simulink model "PassVeh14DOF"  (R2026b)
settings: Solver=ode23tb  StopTime=inf  FixedStep=.001  RelTol=1e-1  EnableMultiTasking=on
model workspace (MAT data in the model file):
  AlgnTrqCambCompl = [0 0 0 0]
  AlgnTrqSteerCompl = [0 0 0 0]
  AxlIxx = 62.3745166667
  AxlM = 160
  BumpCamber = [0 0 0 0]
  BumpCaster = [0 0 0 0]
  BumpSteer = [0 0 0 0]
  CambVsSteerAng = [0 0 0 0]
  CastVsSteerAng = [0 0 0 0]
  Cps = 2
  Cz = 5565.2246438
  CzWhlAxl = 11490.971257
  DCT_Param : object (value not decoded)
  Downshift_Speeds = [9.5625 12.9375 16.3125 19.6875 23.0625 26.4375 29.8125 33.1875 36.5625 39.9375 43.3125 46.6875 ... (28 elements, 4x7)]
  F0z = [2886 2907]
  F0zWhlAxl = 2907
  Hmax = 0.25
  Kz = 52451.0065793
  KzWhlAxl = 138031.612078
  LatCambCompl = [0 0 0 0]
  LatSteerCompl = [0 0 0 0]
  LatWhlCtrComplLat = [0 0 0 0]
  LatWhlCtrComplLng = [0  0  0  0; 0  0  0  0]
  LatWhlCtrDisp = [0 0 0 0]
  LngCambCompl = [0  0  0  0; 0  0  0  0]
  LngCastCompl = [0  0  0  0; 0  0  0  0]
  LngSteerCompl = [0  0  0  0; 0  0  0  0]
  LngWhlCtrCompl = [0  0  0  0; 0  0  0  0]
  LngWhlCtrDisp = [0 0 0 0]
  MotRatios = [1 1]
  NCyl = 6
  NrmlWhlFrcOff = [2886 2886 2907 2907]
  NrmlWhlRates = [52.4510065793 52.4510065793 52.4510065793 52.4510065793]
  Pedal_Positions = [0.1 0.4 0.5 0.9]
  Pstd = 101325
  Rair = 287
  RollCamber : object (value not decoded)
  RollCaster : object (value not decoded)
  RollSteer : object (value not decoded)
  RollStiffArb = [0 0]
  RollStiffArbFrnt = 800
  RollStiffNoArb = [0 0]
  RollStiffNoArbFrnt = 0
  RollStiffNoTwstRear = 0
  ShckFrcVsCompRate = [5.5652246438 5.5652246438 5.5652246438 5.5652246438]
  StatCamber = [0 0 0 0]
  StatCaster = [0 0 0 0]
  StatLdWhlR = [0.3 0.3 0.3 0.3]
  StatToe = [0 0 0 0]
  Trans : object (value not decoded)
  Tstd = 293.15
  Upshift_Speeds = [12.9375 16.3125 19.6875 33 26.4375 29.8125 33.1875 52.5 39.9375 43.3125 46.6875 77.25 ... (28 elements, 4x7)]
  VEH : object (value not decoded)
  Vd = 0.00346
  VrtLdTrnsfr = [0 0 0 0]
  WH : Mass (value not decoded)
  dt3D = 0.05
  f_air = [0 0 0 0 0 0 0 0 0 0 0 0 ... (256 elements, 16x16)]
  f_co = [0 0 0 0 0 0 0 0 0 0 0 0 ... (256 elements, 16x16)]
  f_co2 = [0 0 0 0 0 0 0 0 0 0 0 0 ... (256 elements, 16x16)]
  f_eff = [352.135682859 352.135682859 320.724378192 303.655312657 295.930136708 291.240087194 291.240271258 291.240312459 291.240275452 291.240198499 291.240100781 291.240018769 ... (256 elements, 16x16)]
  f_fuel = [0 0 0 0 0 0 0 0 0 0 0 0 ... (256 elements, 16x16)]
  f_hc = [0 0 0 0 0 0 0 0 0 0 0 0 ... (256 elements, 16x16)]
  f_nox = [0 0 0 0 0 0 0 0 0 0 0 0 ... (256 elements, 16x16)]
  f_pm = [0 0 0 0 0 0 0 0 0 0 0 0 ... (256 elements, 16x16)]
  f_susp_axl_bp = [1 2]
  f_susp_dz_bp = [-0.325022776267 -0.315022776267 -0.305022776267 -0.205022776267 -0.105022776267 -0.00502277626717 0.0949772237328 0.194977223733 0.204977223733 0.214977223733]
  f_susp_dzdot_bp = [-3 -0.3 -0.2 -0.1 0 0.1 0.2 0.3 3]
  f_susp_fmz = [-144070.391448 -93629.24037 -75929.1118915 -20630.5828179 -15385.48216 -10140.3815021 -4895.28084414 349.819813785 -31916.3973792 18437.6709544 -83996.1993354 -33555.0482577 ... (43920 elements, 10x9x61x2x4)]
  f_susp_geom = [0 0 0 0 0 0 0 0 0 0 0 0 ... (3660 elements, 10x61x2x3)]
  f_susp_strgdelta_bp = [-0.523598775598 -0.506145483078 -0.488692190558 -0.471238898038 -0.453785605519 -0.436332312999 -0.418879020479 -0.401425727959 -0.383972435439 -0.366519142919 -0.349065850399 -0.331612557879 ... (61 elements, 1x61)]
  f_tbrake = [0 76.8593923996 105.140482948 131.533638111 157.926793274 176.658631717 176.65727296 176.656856686 176.656879077 176.657093756 176.657404516 176.65772406 ... (256 elements, 16x16)]
  f_tbrake_n_bpt = [0 649.519052838 912.419621844 1175.32019085 1438.22075986 1701.12132886 1964.02189787 2226.92246687 2489.82303588 2752.72360489 3015.62417389 3278.5247429 ... (16 elements, 1x16)]
  f_tbrake_t_bpt = [0 34.6410161514 61.0341713143 87.4273264773 113.82048164 140.213636803 166.606791966 192.999947129 219.393102292 245.786257455 272.179412618 298.572567781 ... (16 elements, 1x16)]
  f_texh = [766.752464599 766.752464599 786.17542386 801.679939032 884.591982581 910.574397722 910.571871054 910.570774534 910.570601632 910.570821151 910.571247242 910.571639815 ... (256 elements, 16x16)]
  f_twc_eff_co = [0.17 0.25 0.45 0.99 0.99 0.99 0.99]
  f_twc_eff_hc = [0.21 0.375 0.75 0.98 0.98 0.98 0.98]
  f_twc_eff_lam = [0.909090909 0.944055944 0.979020979 1 1.013986014 1.048951049 1.083916084]
  f_twc_eff_nox = [0.98 0.98 0.98 0.97 0.05 0.02 0]
  numWheel = 4
symbols that are objects in the model workspace (value not decoded): VEH
libraries: vehdynlibtire x12, vehdynlibsuspension x8, autolibutils x5, sharedtransform x5, shared6dof x2, vehdynlibeom x1, vehdynlibtirecommon x1, matrix_library x1
(part 4 of 9)

== system PassVeh14DOF/Vehicle/Suspension to Chasiss Transforms/Susp2Body ==
  DCM : Inport
  VehAng : Inport  Port=2
  SuspAng : Inport  Port=3
  Fs : Inport  Port=4  Partition=on  PartitionDimension=2  PartitionWidth=1  PartitionOffset=0
  Ms : Inport  Port=5  Partition=on  PartitionDimension=2  PartitionWidth=1  PartitionOffset=0
  For Each : ForEach  DisableCoverage=on
  Inertial to Body : Product  Multiplication=Matrix(*)  InputSameDT=on  SaturateOnIntegerOverflow=on  OutDataTypeStr=Inherit: Same as first input
  Inertial to Body1 : Product  Multiplication=Matrix(*)  InputSameDT=on  SaturateOnIntegerOverflow=on  OutDataTypeStr=Inherit: Same as first input
  Reshape : Reshape
  Reshape1 : Reshape
  Rotation Angles to Direction Cosine Matrix : sharedtransform/Rotation Angles to Direction Cosine Matrix  rotationOrder=ZYX  aMode=2
  Selector : Selector  InputPortWidth=3  IndexOptions=Index vector (dialog)  Indices=[3 2 1]  OutputSizes=1
  Selector1 : Selector  InputPortWidth=3  IndexOptions=Index vector (dialog)  Indices=[1 2]  OutputSizes=1
  Selector2 : Selector  InputPortWidth=3  IndexOptions=Index vector (dialog)  Indices=[3]  OutputSizes=1
  Transpose : Math  Operator=transpose  SignedPower=on
  Unary Minus : UnaryMinus
  Vector Concatenate : Concatenate
  "transform to Inertial axes " : shared6dof/6DOF (Euler Angles)/transform to Inertial axes   SystemSampleTime=-1  VariantActivationTime=update diagram  EmptyChoice=off  PassThrough=off  PassThroughVariantControl=(default)  EmptyChoiceVariantControl=(default)  AllowFlexibleInterface=on  Latency=0  AutoFrameSizeCalculation=off
  transform to Inertial axes 1 : shared6dof/6DOF (Euler Angles)/transform to Inertial axes   SystemSampleTime=-1  VariantActivationTime=update diagram  EmptyChoice=off  PassThrough=off  PassThroughVariantControl=(default)  EmptyChoiceVariantControl=(default)  AllowFlexibleInterface=on  Latency=0  AutoFrameSizeCalculation=off
  FsB : Outport  ConcatenationDimension=2  VectorParamsAs1DForOutWhenUnconnected=off
  MsB : Outport  Port=2  ConcatenationDimension=2  VectorParamsAs1DForOutWhenUnconnected=off
  wires:
  Reshape/1 -> Inertial to Body/2
  Inertial to Body/1 -> FsB/1
  SuspAng/1 -> Unary Minus/1
  Selector/1 -> Rotation Angles to Direction Cosine Matrix/1
  Fs/1 -> "transform to Inertial axes "/1
  Transpose/1 -> transform to Inertial axes 1/2, "transform to Inertial axes "/2
  Rotation Angles to Direction Cosine Matrix/1 -> Transpose/1
  "transform to Inertial axes "/1 -> Reshape/1
  transform to Inertial axes 1/1 -> Reshape1/1
  Inertial to Body1/1 -> MsB/1
  Reshape1/1 -> Inertial to Body1/2
  DCM/1 -> Inertial to Body1/1, Inertial to Body/1
  Ms/1 -> transform to Inertial axes 1/1
  VehAng/1 -> Selector2/1
  Unary Minus/1 -> Selector1/1
  Selector1/1 -> Vector Concatenate/1
  Vector Concatenate/1 -> Selector/1
  Selector2/1 -> Vector Concatenate/2

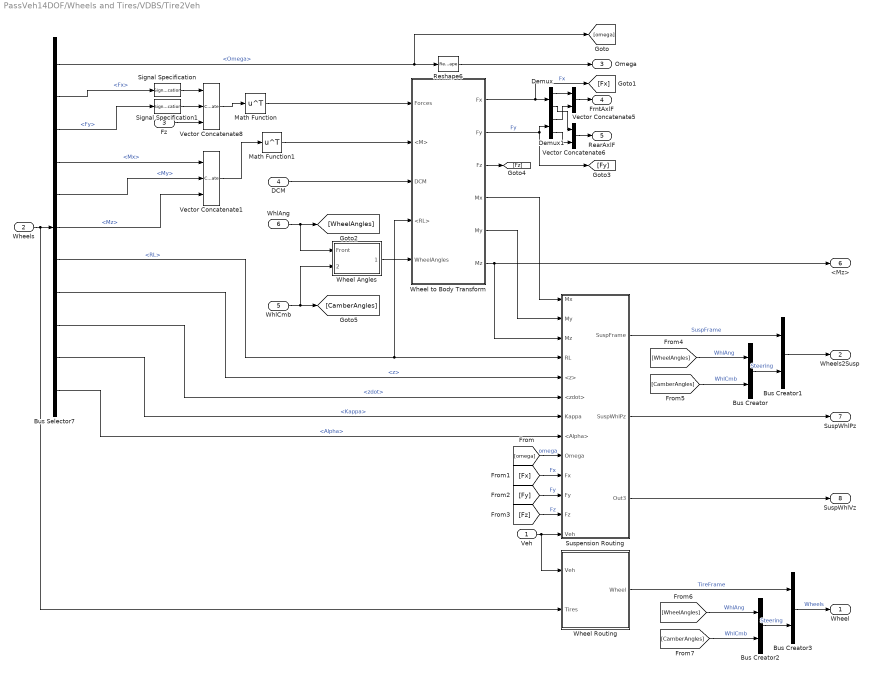
== system PassVeh14DOF/Wheels and Tires/VDBS/Tire2Veh ==
  Veh : Inport
  Wheels : Inport  Port=2
  Fz : Inport  Port=3  PortDimensions=4
  DCM : Inport  Port=4
  WhlCmb : Inport  Port=5
  WhlAng : Inport  Port=6
  Bus Creator{,1..3} (4 alike) : BusCreator  Inputs=2
  Bus Selector7 : BusSelector  OutputSignals=Omega,Fx,Fy,Mx,My,Mz,RL,z,zdot,Kappa,Alpha
  Demux : Demux  Outputs=[2,2]
  Demux1 : Demux  Outputs=[2,2]
  Math Function : Math  Operator=transpose  SignedPower=on
  Math Function1 : Math  Operator=transpose  SignedPower=on
  Reshape6 : Reshape  OutputDimensionality=Customize  OutputDimensions=[2,2]
  Signal Specification : SignalSpecification  Dimensions=4
  Signal Specification1 : SignalSpecification  Dimensions=4
  Suspension Routing : Subsystem
  Vector Concatenate1 : Concatenate  NumInputs=3  Mode=Multidimensional array  ConcatenateDimension=2
  Vector Concatenate5 : Concatenate  Mode=Multidimensional array  ConcatenateDimension=2
  Vector Concatenate6 : Concatenate  Mode=Multidimensional array  ConcatenateDimension=2
  Vector Concatenate8 : Concatenate  NumInputs=3  Mode=Multidimensional array  ConcatenateDimension=2
  Wheel Angles : Subsystem
  Wheel Routing : Subsystem
  Wheel to Body Transform : Subsystem
  Wheel : Outport  VectorParamsAs1DForOutWhenUnconnected=off
  Wheels2Susp : Outport  Port=2  VectorParamsAs1DForOutWhenUnconnected=off
  Omega : Outport  Port=3  VectorParamsAs1DForOutWhenUnconnected=off
  FrntAxlF : Outport  Port=4  VectorParamsAs1DForOutWhenUnconnected=off
  RearAxlF : Outport  Port=5  VectorParamsAs1DForOutWhenUnconnected=off
  <Mz> : Outport  Port=6  VectorParamsAs1DForOutWhenUnconnected=off
  SuspWhlPz : Outport  Port=7  VectorParamsAs1DForOutWhenUnconnected=off
  SuspWhlVz : Outport  Port=8  VectorParamsAs1DForOutWhenUnconnected=off
  wires:
  Fz/1 -> Vector Concatenate8/3
  Vector Concatenate6/1 -> RearAxlF/1
  Vector Concatenate8/1 -> Math Function/1
  Demux/2 -> Vector Concatenate6/1
  Demux1/2 -> Vector Concatenate6/2
  Demux/1 -> Vector Concatenate5/1
  Math Function/1 -> Wheel to Body Transform/1(Forces)
  Bus Selector7/2 -> Signal Specification/1  "<Fx>"
  Vector Concatenate5/1 -> FrntAxlF/1
  Wheels/1 -> Wheel Routing/2(Tires), Bus Selector7/1
  Reshape6/1 -> Omega/1
  Demux1/1 -> Vector Concatenate5/2
  Wheel Angles/1(Vehicle) -> Wheel to Body Transform/5(WheelAngles)
  Bus Selector7/1 -> [omega], Reshape6/1  "<Omega>"
  WhlAng/1 -> Wheel Angles/1(Front), [WheelAngles]
  Wheel to Body Transform/3(Fz) -> [Fz]
  WhlCmb/1 -> Wheel Angles/2(Camber), [CamberAngles]
  Bus Selector7/3 -> Signal Specification1/1  "<Fy>"
  Bus Selector7/5 -> Vector Concatenate1/2  "<My>"
  [omega] -> Suspension Routing/9(Omega)  "omega"
  [Fx] -> Suspension Routing/10(Fx)  "Fx"
  Bus Selector7/8 -> Suspension Routing/5(<z>)  "<z>"
  [Fy] -> Suspension Routing/11(Fy)  "Fy"
  [Fz] -> Suspension Routing/12(Fz)  "Fz"
  Bus Selector7/9 -> Suspension Routing/6(<zdot>)  "<zdot>"
  Bus Selector7/10 -> Suspension Routing/7(Kappa)  "<Kappa>"
  Suspension Routing/2(SuspWhlPz) -> SuspWhlPz/1
  Suspension Routing/3(Out3) -> SuspWhlVz/1
  [WheelAngles] -> Bus Creator/1  "WhlAng"
  Bus Creator1/1 -> Wheels2Susp/1
  Suspension Routing/1(SuspFrame) -> Bus Creator1/1  "SuspFrame"
  [CamberAngles] -> Bus Creator/2  "WhlCmb"
  Bus Creator/1 -> Bus Creator1/2  "Steering"
  Bus Selector7/11 -> Suspension Routing/8(<Alpha>)  "<Alpha>"
  Wheel to Body Transform/1(Fx) -> [Fx], Demux/1  "Fx"
  Wheel to Body Transform/2(Fy) -> [Fy], Demux1/1  "Fy"
  Veh/1 -> Wheel Routing/1(Veh), Suspension Routing/13(Veh)
  Signal Specification/1 -> Vector Concatenate8/1
  Signal Specification1/1 -> Vector Concatenate8/2
  Wheel Routing/1(Wheel) -> Bus Creator3/1  "TireFrame"
  Bus Creator2/1 -> Bus Creator3/2  "Steering"
  [CamberAngles] -> Bus Creator2/2  "WhlCmb"
  Bus Creator3/1 -> Wheel/1  "Wheels"
  [WheelAngles] -> Bus Creator2/1  "WhlAng"
  Bus Selector7/4 -> Vector Concatenate1/1  "<Mx>"
  Bus Selector7/6 -> Vector Concatenate1/3  "<Mz>"
  Vector Concatenate1/1 -> Math Function1/1
  DCM/1 -> Wheel to Body Transform/3(DCM)
  Wheel to Body Transform/4(Mx) -> Suspension Routing/1(Mx)
  Wheel to Body Transform/5(My) -> Suspension Routing/2(My)
  Wheel to Body Transform/6(Mz) -> Suspension Routing/3(Mz), <Mz>/1
  Math Function1/1 -> Wheel to Body Transform/2(<M>)
  Bus Selector7/7 -> Wheel to Body Transform/4(<RL>), Suspension Routing/4(RL)  "<RL>"

== system PassVeh14DOF/Wheels and Tires/VDBS/Tires ==
  "DriveTorque " : Inport
  "Brake Pressure " : Inport  Port=2
  "r " : Inport  Port=3
  "Vx " : Inport  Port=4
  "Vy " : Inport  Port=5
  "Camber " : Inport  Port=6
  "Press " : Inport  Port=7
  "lambda " : Inport  Port=8
  "Gnd " : Inport  Port=9
  "FzSusp " : Inport  Port=10
  Dugoff Tires Vector : Subsystem  VariantControl=4
  Fiala Tires : Subsystem  VariantControl=1
  Fiala Tires Vector : Subsystem  VariantControl=3
  MF Tires : Subsystem  VariantControl=0
  MF Tires Vector : Subsystem  VariantControl=2
  " Wheels" : Outport  VectorParamsAs1DForOutWhenUnconnected=off

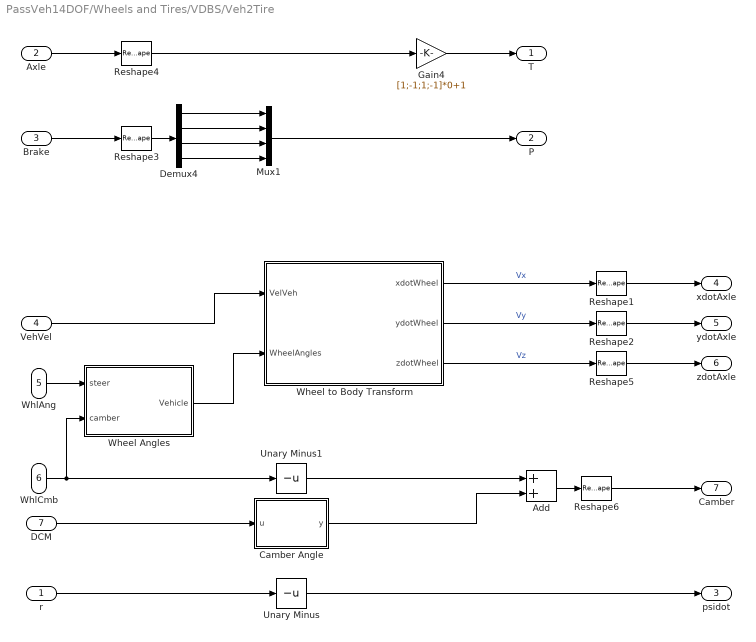
== system PassVeh14DOF/Wheels and Tires/VDBS/Veh2Tire ==
  r : Inport
  Axle : Inport  Port=2
  Brake : Inport  Port=3
  VehVel : Inport  Port=4
  WhlAng : Inport  Port=5
  WhlCmb : Inport  Port=6
  DCM : Inport  Port=7
  Add : Sum
  Camber Angle : MATLAB Function  TreatAsAtomicUnit=on
  Demux4 : Demux
  Gain4 : Gain  Gain=[1;-1;1;-1]*0+1
  Mux1 : Mux
  Reshape{1..6} (6 alike) : Reshape
  Unary Minus : UnaryMinus
  Unary Minus1 : UnaryMinus
  Wheel Angles : Subsystem
  Wheel to Body Transform : Subsystem
  T : Outport  Unit=N*m  VectorParamsAs1DForOutWhenUnconnected=off
  P : Outport  Port=2  Unit=Pa  VectorParamsAs1DForOutWhenUnconnected=off
  psidot : Outport  Port=3  Unit=rad/s  VectorParamsAs1DForOutWhenUnconnected=off
  xdotAxle : Outport  Port=4  Unit=m/s  VectorParamsAs1DForOutWhenUnconnected=off
  ydotAxle : Outport  Port=5  Unit=m/s  VectorParamsAs1DForOutWhenUnconnected=off
  zdotAxle : Outport  Port=6  Unit=m/s  VectorParamsAs1DForOutWhenUnconnected=off
  Camber : Outport  Port=7  Unit=rad  VectorParamsAs1DForOutWhenUnconnected=off
  wires:
  Demux4/1 -> Mux1/1
  Brake/1 -> Reshape3/1
  Demux4/4 -> Mux1/4
  Axle/1 -> Reshape4/1
  Wheel to Body Transform/1(xdotWheel) -> Reshape1/1  "Vx"
  Demux4/2 -> Mux1/2
  Wheel to Body Transform/2(ydotWheel) -> Reshape2/1  "Vy"
  WhlAng/1 -> Wheel Angles/1(steer)
  Mux1/1 -> P/1
  r/1 -> Unary Minus/1
  Demux4/3 -> Mux1/3
  Reshape3/1 -> Demux4/1
  Gain4/1 -> T/1
  Reshape4/1 -> Gain4/1
  VehVel/1 -> Wheel to Body Transform/1(VelVeh)
  Wheel to Body Transform/3(zdotWheel) -> Reshape5/1  "Vz"
  WhlCmb/1 -> Unary Minus1/1, Wheel Angles/2(camber)
  Unary Minus/1 -> psidot/1
  Wheel Angles/1(Vehicle) -> Wheel to Body Transform/2(WheelAngles)
  Reshape1/1 -> xdotAxle/1
  Reshape2/1 -> ydotAxle/1
  Reshape5/1 -> zdotAxle/1
  Unary Minus1/1 -> Add/1
  DCM/1 -> Camber Angle/1(u)
  Add/1 -> Reshape6/1
  Camber Angle/1(y) -> Add/2
  Reshape6/1 -> Camber/1

== system PassVeh14DOF/Suspension/Kinematics and Compliance Independent Suspension/Calculate dynamic track width from lateral wheel center displacement change/Front Track Calculation ==
  dWhlY : Inport
  sign : Inport  Port=2
  Abs : Abs  ZeroCross=off  SaturateOnIntegerOverflow=off
  Abs1 : Abs  ZeroCross=off  SaturateOnIntegerOverflow=off
  Add : Sum  Inputs=+++
  Front Left select : Selector  InputPortWidth=4  IndexOptions=Index vector (dialog)  Indices=1  OutputSizes=1
  Front Left select1 : Selector  InputPortWidth=4  IndexOptions=Index vector (dialog)  Indices=1  OutputSizes=1
  Front Right select : Selector  InputPortWidth=4  IndexOptions=Index vector (dialog)  Indices=2  OutputSizes=1
  Front Right select1 : Selector  InputPortWidth=4  IndexOptions=Index vector (dialog)  Indices=2  OutputSizes=1
  Front Track : Constant  Value=w(1)
  Product : Product
  Product1 : Product
  w_front : Outport
  wires:
  Front Track/1 -> Add/1
  Front Left select/1 -> Abs/1
  Front Right select/1 -> Abs1/1
  sign/1 -> Front Right select1/1, Front Left select1/1
  Product/1 -> Add/2
  Front Left select1/1 -> Product/2
  Abs1/1 -> Product1/1
  Abs/1 -> Product/1
  Product1/1 -> Add/3
  Front Right select1/1 -> Product1/2
  Add/1 -> w_front/1
  dWhlY/1 -> Front Right select/1, Front Left select/1

== system PassVeh14DOF/Suspension/Kinematics and Compliance Independent Suspension/Calculate dynamic track width from lateral wheel center displacement change/Rear Track Calculation ==
  dWhlY : Inport
  sign : Inport  Port=2
  Abs2 : Abs  ZeroCross=off  SaturateOnIntegerOverflow=off
  Abs3 : Abs  ZeroCross=off  SaturateOnIntegerOverflow=off
  Add1 : Sum  Inputs=+++
  Product2 : Product
  Product3 : Product
  Rear Left select : Selector  InputPortWidth=4  IndexOptions=Index vector (dialog)  Indices=3  OutputSizes=1
  Rear Left select1 : Selector  InputPortWidth=4  IndexOptions=Index vector (dialog)  Indices=3  OutputSizes=1
  Rear Right select : Selector  InputPortWidth=4  IndexOptions=Index vector (dialog)  Indices=4  OutputSizes=1
  Rear Right select1 : Selector  InputPortWidth=4  IndexOptions=Index vector (dialog)  Indices=4  OutputSizes=1
  Rear Track : Constant  Value=w(2)
  w_rear : Outport
  wires:
  Product2/1 -> Add1/2
  Abs2/1 -> Product2/1
  Rear Left select/1 -> Abs2/1
  Rear Left select1/1 -> Product2/2
  Rear Right select1/1 -> Product3/2
  Abs3/1 -> Product3/1
  dWhlY/1 -> Rear Left select/1, Rear Right select/1
  sign/1 -> Rear Right select1/1, Rear Left select1/1
  Rear Right select/1 -> Abs3/1
  Rear Track/1 -> Add1/1
  Product3/1 -> Add1/3
  Add1/1 -> w_rear/1

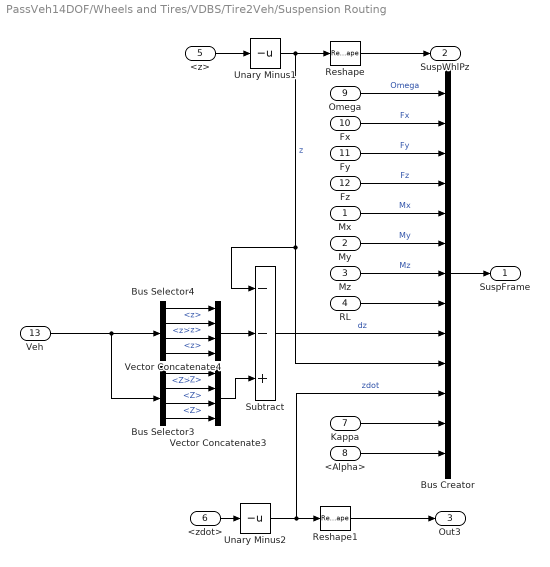
== system PassVeh14DOF/Wheels and Tires/VDBS/Tire2Veh/Suspension Routing ==
  Mx : Inport
  My : Inport  Port=2
  Mz : Inport  Port=3
  RL : Inport  Port=4
  <z> : Inport  Port=5
  <zdot> : Inport  Port=6
  Kappa : Inport  Port=7
  <Alpha> : Inport  Port=8
  Omega : Inport  Port=9
  Fx : Inport  Port=10
  Fy : Inport  Port=11
  Fz : Inport  Port=12
  Veh : Inport  Port=13
  Bus Creator : BusCreator  Inputs=13
  Bus Selector3 : BusSelector  OutputSignals=InertFrm.FrntAxl.Lft.Disp.Z,InertFrm.FrntAxl.Rght.Disp.Z,InertFrm.RearAxl.Lft.Disp.Z,InertFrm.RearAxl.Rght.Disp.Z
  Bus Selector4 : BusSelector  OutputSignals=BdyFrm.FrntAxl.Lft.Disp.z,BdyFrm.FrntAxl.Rght.Disp.z,BdyFrm.RearAxl.Lft.Disp.z,BdyFrm.RearAxl.Rght.Disp.z
  Reshape : Reshape  OutputDimensionality=Row vector (2-D)
  Reshape1 : Reshape  OutputDimensionality=Row vector (2-D)
  Subtract : Sum  Inputs=--+
  Unary Minus1 : UnaryMinus
  Unary Minus2 : UnaryMinus
  Vector Concatenate3 : Concatenate  NumInputs=4
  Vector Concatenate4 : Concatenate  NumInputs=4
  SuspFrame : Outport  VectorParamsAs1DForOutWhenUnconnected=off
  SuspWhlPz : Outport  Port=2  VectorParamsAs1DForOutWhenUnconnected=off
  Out3 : Outport  Port=3  VectorParamsAs1DForOutWhenUnconnected=off
  wires:
  RL/1 -> Bus Creator/8
  Unary Minus1/1 -> Bus Creator/10, Subtract/1, Reshape/1  "z"
  Fz/1 -> Bus Creator/4  "Fz"
  <zdot>/1 -> Unary Minus2/1
  Mz/1 -> Bus Creator/7  "Mz"
  Unary Minus2/1 -> Bus Creator/11, Reshape1/1  "zdot"
  <z>/1 -> Unary Minus1/1
  Bus Creator/1 -> SuspFrame/1
  Fy/1 -> Bus Creator/3  "Fy"
  Omega/1 -> Bus Creator/1  "Omega"
  Fx/1 -> Bus Creator/2  "Fx"
  Reshape1/1 -> Out3/1
  Kappa/1 -> Bus Creator/12
  Reshape/1 -> SuspWhlPz/1
  Mx/1 -> Bus Creator/5  "Mx"
  My/1 -> Bus Creator/6  "My"
  <Alpha>/1 -> Bus Creator/13
  Veh/1 -> Bus Selector3/1, Bus Selector4/1
  Bus Selector3/4 -> Vector Concatenate3/4  "<Z>"
  Subtract/1 -> Bus Creator/9  "dz"
  Bus Selector4/1 -> Vector Concatenate4/1  "<z>"
  Bus Selector3/1 -> Vector Concatenate3/1  "<Z>"
  Vector Concatenate3/1 -> Subtract/3
  Vector Concatenate4/1 -> Subtract/2
  Bus Selector4/2 -> Vector Concatenate4/2  "<z>"
  Bus Selector3/3 -> Vector Concatenate3/3  "<Z>"
  Bus Selector3/2 -> Vector Concatenate3/2  "<Z>"
  Bus Selector4/4 -> Vector Concatenate4/4  "<z>"
  Bus Selector4/3 -> Vector Concatenate4/3  "<z>"

== system PassVeh14DOF/Wheels and Tires/VDBS/Tire2Veh/Wheel Angles ==
  Front : Inport
  Camber : Inport  Port=2
  Constant : Constant  Value=zeros(4,1)
  Reshape : Reshape  OutputDimensionality=Row vector (2-D)
  Reshape1 : Reshape  OutputDimensionality=Row vector (2-D)
  Reshape2 : Reshape  OutputDimensionality=Row vector (2-D)
  Vector Concatenate3 : Concatenate  NumInputs=3  Mode=Multidimensional array
  Vehicle : Outport  VectorParamsAs1DForOutWhenUnconnected=off
  wires:
  Reshape/1 -> Vector Concatenate3/3
  Reshape2/1 -> Vector Concatenate3/2
  Vector Concatenate3/1 -> Vehicle/1
  Reshape1/1 -> Vector Concatenate3/1
  Front/1 -> Reshape/1
  Camber/1 -> Reshape1/1
  Constant/1 -> Reshape2/1

== system PassVeh14DOF/Wheels and Tires/VDBS/Tire2Veh/Wheel Routing ==
  Veh : Inport
  Tires : Inport  Port=2
  Bus Creator : BusCreator  Inputs=13
  Bus Selector : BusSelector  OutputSignals=Omega,Fx,Fy,Fz,Mx,My,Mz,Re,z,zdot,Kappa,Alpha
  Bus Selector3 : BusSelector  OutputSignals=InertFrm.FrntAxl.Lft.Disp.Z,InertFrm.FrntAxl.Rght.Disp.Z,InertFrm.RearAxl.Lft.Disp.Z,InertFrm.RearAxl.Rght.Disp.Z
  Bus Selector4 : BusSelector  OutputSignals=BdyFrm.FrntAxl.Lft.Disp.z,BdyFrm.FrntAxl.Rght.Disp.z,BdyFrm.RearAxl.Lft.Disp.z,BdyFrm.RearAxl.Rght.Disp.z
  Subtract : Sum  Inputs=-+-
  Vector Concatenate3 : Concatenate  NumInputs=4
  Vector Concatenate4 : Concatenate  NumInputs=4
  Wheel : Outport  VectorParamsAs1DForOutWhenUnconnected=off
  wires:
  Bus Selector4/3 -> Vector Concatenate4/3  "<z>"
  Bus Selector4/4 -> Vector Concatenate4/4  "<z>"
  Bus Selector3/2 -> Vector Concatenate3/2  "<Z>"
  Bus Selector3/3 -> Vector Concatenate3/3  "<Z>"
  Bus Selector4/2 -> Vector Concatenate4/2  "<z>"
  Vector Concatenate4/1 -> Subtract/2
  Vector Concatenate3/1 -> Subtract/3
  Bus Selector3/1 -> Vector Concatenate3/1  "<Z>"
  Bus Selector4/1 -> Vector Concatenate4/1  "<z>"
  Subtract/1 -> Bus Creator/9  "dz"
  Bus Selector3/4 -> Vector Concatenate3/4  "<Z>"
  Veh/1 -> Bus Selector4/1, Bus Selector3/1
  Bus Selector/12 -> Bus Creator/13  "<Alpha>"
  Bus Selector/6 -> Bus Creator/6  "<My>"
  Bus Selector/5 -> Bus Creator/5  "<Mx>"
  Bus Selector/11 -> Bus Creator/12  "<Kappa>"
  Bus Selector/2 -> Bus Creator/2  "<Fx>"
  Bus Selector/1 -> Bus Creator/1  "<Omega>"
  Bus Selector/3 -> Bus Creator/3  "<Fy>"
  Bus Creator/1 -> Wheel/1
  Bus Selector/10 -> Bus Creator/11  "<zdot>"
  Bus Selector/7 -> Bus Creator/7  "<Mz>"
  Bus Selector/4 -> Bus Creator/4  "<Fz>"
  Bus Selector/9 -> Subtract/1, Bus Creator/10  "<z>"
  Tires/1 -> Bus Selector/1  "TireFrame"
  Bus Selector/8 -> Bus Creator/8  "<Re>"

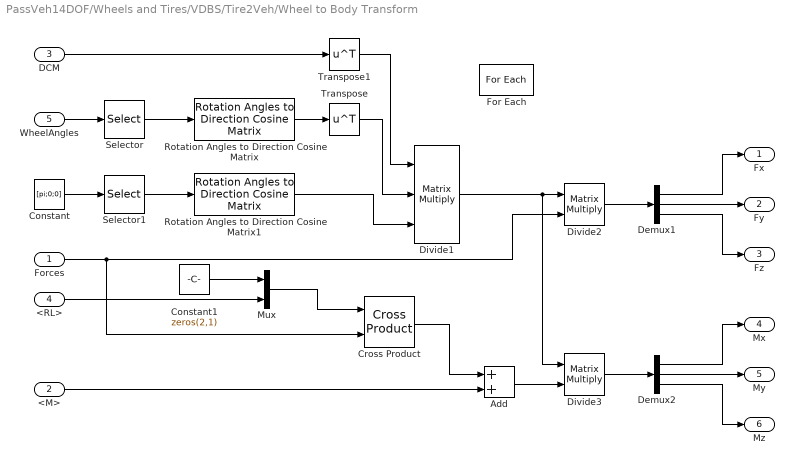
== system PassVeh14DOF/Wheels and Tires/VDBS/Tire2Veh/Wheel to Body Transform ==
  Forces : Inport  PortDimensions=[3,1]  Partition=on  PartitionDimension=2  PartitionWidth=1  PartitionOffset=0
  <M> : Inport  Port=2  PortDimensions=[3,1]  Partition=on  PartitionDimension=2  PartitionWidth=1  PartitionOffset=0
  DCM : Inport  Port=3  Partition=on  PartitionDimension=3  PartitionWidth=1  PartitionOffset=0
  <RL> : Inport  Port=4  Partition=on  PartitionDimension=1  PartitionWidth=1  PartitionOffset=0
  WheelAngles : Inport  Port=5  Partition=on  PartitionDimension=2  PartitionWidth=1  PartitionOffset=0
  Add : Sum
  Constant : Constant  Value=[pi;0;0]
  Constant1 : Constant  Value=zeros(2,1)
  Cross Product : matrix_library/Cross Product
  Demux1 : Demux  Outputs=3
  Demux2 : Demux  Outputs=3
  Divide1 : Product  Inputs=***  Multiplication=Matrix(*)
  Divide2 : Product  Inputs=**  Multiplication=Matrix(*)
  Divide3 : Product  Inputs=**  Multiplication=Matrix(*)
  For Each : ForEach  DisableCoverage=on
  Mux : Mux  Inputs=2
  Rotation Angles to Direction Cosine Matrix : sharedtransform/Rotation Angles to Direction Cosine Matrix  rotationOrder=ZYX  aMode=2
  Rotation Angles to Direction Cosine Matrix1 : sharedtransform/Rotation Angles to Direction Cosine Matrix  rotationOrder=ZYX  aMode=2
  Selector : Selector  InputPortWidth=3  IndexOptions=Index vector (dialog)  Indices=[3 2 1]  OutputSizes=1
  Selector1 : Selector  InputPortWidth=3  IndexOptions=Index vector (dialog)  Indices=[3 2 1]  OutputSizes=1
  Transpose : Math  Operator=transpose
  Transpose1 : Math  Operator=transpose
  Fx : Outport  ConcatenationDimension=1  VectorParamsAs1DForOutWhenUnconnected=off
  Fy : Outport  Port=2  ConcatenationDimension=1  VectorParamsAs1DForOutWhenUnconnected=off
  Fz : Outport  Port=3  ConcatenationDimension=1  VectorParamsAs1DForOutWhenUnconnected=off
  Mx : Outport  Port=4  ConcatenationDimension=1  VectorParamsAs1DForOutWhenUnconnected=off
  My : Outport  Port=5  ConcatenationDimension=1  VectorParamsAs1DForOutWhenUnconnected=off
  Mz : Outport  Port=6  ConcatenationDimension=1  VectorParamsAs1DForOutWhenUnconnected=off
  wires:
  Demux1/1 -> Fx/1
  Demux1/2 -> Fy/1
  Demux1/3 -> Fz/1
  Rotation Angles to Direction Cosine Matrix/1 -> Transpose/1
  Forces/1 -> Divide2/2, Cross Product/2
  WheelAngles/1 -> Selector/1
  Selector/1 -> Rotation Angles to Direction Cosine Matrix/1
  Rotation Angles to Direction Cosine Matrix1/1 -> Divide1/3
  Selector1/1 -> Rotation Angles to Direction Cosine Matrix1/1
  Constant/1 -> Selector1/1
  Transpose/1 -> Divide1/2
  DCM/1 -> Transpose1/1
  Transpose1/1 -> Divide1/1
  Divide2/1 -> Demux1/1
  Divide3/1 -> Demux2/1
  Divide1/1 -> Divide3/1, Divide2/1
  <M>/1 -> Add/2
  Demux2/3 -> Mz/1
  Demux2/2 -> My/1
  Demux2/1 -> Mx/1
  Add/1 -> Divide3/2
  Cross Product/1 -> Add/1
  Mux/1 -> Cross Product/1
  <RL>/1 -> Mux/2
  Constant1/1 -> Mux/1
